simulink library "sm_wheel_loader_lib"  (R2025a)
settings: Solver=VariableStepAuto  StartTime=0.0  StopTime=10.0  RelTol=1e-3
undefined symbols (not defined in the file): AToTOrificeVector, BiPOrificeVector, boomHEArea, boomREArea, BToTOrificeVector, fluids, GRake, GToothL, GToothR, HMPST, HydFcnParams, logLoad, Position, PToAOrificeVector, PToBOrificeVector, RakeL, RakeR, testInput, Wheel_Loader, X, Y, Z
libraries: sm_lib x694, fl_lib x183, nesl_utility x74, SimscapeFluids_lib x62, sdl_lib x25, cvt_components_lib x25, simulink_extras x5, $bdroot x4, wheel_loader_contact_lib x4, ee_lib x2, SignalEditorBlockLib x1, batteryecm_lib x1
(part 11 of 26)

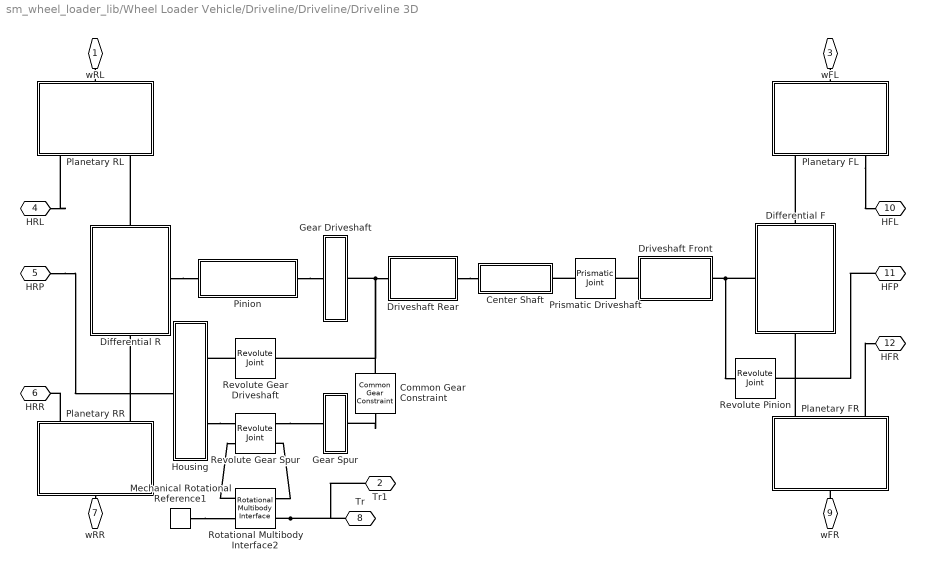
== system sm_wheel_loader_lib/Wheel Loader Vehicle/Driveline/Driveline/Driveline 3D ==
  Center Shaft : Subsystem
      mask Display: image('sm_wheel_loader_driveline_centerShaft_IMAGE.png');
  Common Gear Constraint : sm_lib/Gears and Couplings/Gears/Common Gear Constraint  GearType=External  SpecificationType=CenterDistanceRatio  CenterDistance=0.159173333333337  CenterDistanceUnits=m  GearRatio=60/34  BaseGearRadius=10.0  BaseGearRadiusUnits=cm  FollGearRadius=10.0  FollGearRadiusUnits=cm
  Differential F : Subsystem  mask{diff_casing_opc=HMPST.Vis.FDiffHou.opc}
      mask prompts: diff_casing_opc "Differential Casing Opacity (0-1)"
      settings: PortSchema="{\"entries\":[{\"content\":{\"sides\":[{\"content\":{\"connectorIds\":[\"LConn1\"]},\"type\":\"ConnectorPlacement.EquallySpacedRectSide\",\"uuid\":\"6caa8627-c586-4624-9941-b1de02eaac8c\"},{\"content\":{\"side\":\"RIGHT\"},\"type\":\"ConnectorPlacement.EquallySpacedRectSide\",\"uuid\":\"92f56e30-b0a7-4c10-9542-dd710977b4de\"},{\"content\":{\"connectorIds\":[\"LConn2\"],\"side\":\"TOP\"},\"type\":\"ConnectorPlacement.EquallySpacedRectSide\",\"uuid\":\"6e0658b9-6e92-4387-ac01-d2f307bfa341\"},{\"content\":{\"connectorIds\":[\"RConn1\"],\"side\":\"BOTTOM\"},\"type\":\"ConnectorPlacement.EquallySpacedRectSide\",\"uuid\":\"3080ce9a-db32-4b14-9c1c-37c42147fc35\"}]},\"type\":\"ConnectorPlacement.EquallySpacedConnector\",\"uuid\":\"9cd5bcd7-248c-4c6f-ba2a-fbf4d8f64778\"}],\"packageUris\":[\"http://schema.mathworks.com/mf0/Connector/R2020b\"],\"version\":\"1.0\"}"
      mask Display: image('sm_wheel_loader_Driveline3D_FDiff_IMAGE.png');
  Differential R : Subsystem  mask{diffR_casing_opc=HMPST.Vis.RDiffHou.opc}
      mask prompts: diffR_casing_opc "Differential Casing Opacity"
      settings: PortSchema="{\"entries\":[{\"content\":{\"sides\":[{\"content\":{\"connectorIds\":[\"LConn1\"]},\"type\":\"ConnectorPlacement.EquallySpacedRectSide\",\"uuid\":\"c6c34cb6-4adc-4dcc-9206-ba657dac7b98\"},{\"content\":{\"connectorIds\":[\"RConn1\"],\"side\":\"RIGHT\"},\"type\":\"ConnectorPlacement.EquallySpacedRectSide\",\"uuid\":\"746b050e-ecd9-4d25-a3bf-d6d079e98d03\"},{\"content\":{\"side\":\"TOP\"},\"type\":\"ConnectorPlacement.EquallySpacedRectSide\",\"uuid\":\"a331b284-bfab-47fb-9050-1886c295eab8\"},{\"content\":{\"connectorIds\":[\"RConn2\"],\"side\":\"BOTTOM\"},\"type\":\"ConnectorPlacement.EquallySpacedRectSide\",\"uuid\":\"57ab5774-feb0-4c3e-8c1c-741aef2b477c\"}]},\"type\":\"ConnectorPlacement.EquallySpacedConnector\",\"uuid\":\"0234f3ec-52d5-4d95-88b5-4fa84eea842c\"}],\"packageUris\":[\"http://schema.mathworks.com/mf0/Connector/R2020b\"],\"version\":\"1.0\"}"
      mask Display: image('sm_wheel_loader_Driveline3D_RDiff_IMAGE.png');
  Driveshaft Front : Subsystem  mask{popup_driveJointF=CV Joint}
      mask prompts: popup_driveJointF "Joint Type"
      mask init:
      | if(strcmp(get_param(gcb,'popup_driveJointF'),'CV Joint'))
      |     set_param([gcb '/Joint'],'LabelModeActiveChoice','CV_Joint');
      | else
      |     set_param([gcb '/Joint'],'LabelModeActiveChoice','U_Joint');
      | end
      settings: AttributesFormatString=%<popup_driveJointF>
      mask TypeOptions popup_driveJointF: CV Joint | U Joint
      mask Display:
      | if(strcmp(get_param(gcb,'popup_driveJointF'),'U Joint'))
      |     image('sm_wheel_loader_driveline_ujointF_IMAGE.png');
      | elseif(strcmp(get_param(gcb,'popup_driveJointF'),'CV Joint'))
      |     image('sm_wheel_loader_driveline_cvjointF_IMAGE.png');
      | end
  Driveshaft Rear : Subsystem  mask{popup_driveJointR=CV Joint}
      mask prompts: popup_driveJointR "Joint Type"
      mask init:
      | if(strcmp(get_param(gcb,'popup_driveJointR'),'CV Joint'))
      |     set_param([gcb '/Joint'],'LabelModeActiveChoice','CV_Joint');
      | else
      |     set_param([gcb '/Joint'],'LabelModeActiveChoice','U_Joint');
      | end
      settings: AttributesFormatString=%<popup_driveJointR>
      mask TypeOptions popup_driveJointR: CV Joint | U Joint
      mask Display:
      | if(strcmp(get_param(gcb,'popup_driveJointR'),'U Joint'))
      |     image('sm_wheel_loader_driveline_ujointR_IMAGE.png');
      | elseif(strcmp(get_param(gcb,'popup_driveJointR'),'CV Joint'))
      |     image('sm_wheel_loader_driveline_cvjointR_IMAGE.png');
      | end
  Gear Driveshaft : Subsystem  Tag=431AF5D6-54DA-7142-9431-C4596B630D74
      mask Display: image('sm_wheel_loader_driveline_gearDriveshaft_IMAGE.png')
  Gear Spur : Subsystem  Tag=6EB64544-2A1C-0847-BADC-74C9179BE488
      mask Display: image('sm_wheel_loader_driveline_gearSpur_IMAGE.png')
  Housing : Subsystem  Tag=FD1DF3FF-DA5A-0743-8F9C-61712535B657  mask{finalDr_casing_opc=HMPST.Vis.TfrGearHou.opc}
      mask prompts: finalDr_casing_opc "Final Drive Housing Opacity (0-1)"
      mask Display: image('sm_wheel_loader_driveline_gearHousing_IMAGE.png');
  Mechanical Rotational Reference1 : fl_lib/Mechanical/Rotational Elements/Mechanical Rotational Reference
  Pinion : Subsystem  Tag=8E104B94-12D7-814C-ADF4-87AC864C83F8
      mask Display: image('sm_wheel_loader_driveline_pinionR_IMAGE.png');
  Planetary FL : Subsystem  mask{casing_opc=HMPST.Vis.WhlPlaHou.opc}
      mask prompts: casing_opc "Casing Opacity (0-1)"
      mask Display: image('sm_wheel_loader_driveline_planetaryHubLtrans_IMAGE.png');
  Planetary FR : Subsystem  mask{casing_opc=HMPST.Vis.WhlPlaHou.opc}
      mask prompts: casing_opc "Casing Opacity (0-1)"
      mask Display: image('sm_wheel_loader_driveline_planetaryHubRtrans_IMAGE.png');
  Planetary RL : Subsystem  mask{casing_opc=HMPST.Vis.WhlPlaHou.opc}
      mask prompts: casing_opc "Casing Opacity (0-1)"
      mask Display: image('sm_wheel_loader_driveline_planetaryHubLtrans_IMAGE.png');
  Planetary RR : Subsystem  mask{casing_opc=HMPST.Vis.WhlPlaHou.opc}
      mask prompts: casing_opc "Casing Opacity (0-1)"
      mask Display: image('sm_wheel_loader_driveline_planetaryHubRtrans_IMAGE.png');
  Prismatic Driveshaft : sm_lib/Joints/Prismatic Joint  JointMode=Normal  CompositeWrenchDir=FollowerOnBase  CompositeWrenchFrame=BaseFrame  SenseConstraintForce=off  SenseConstraintTorque=off  SenseTotalForce=off  SenseTotalTorque=off  PositionTargetSpecify=off  PositionTargetPriority=High  PositionTargetValue=0  PositionTargetValueUnits=m  VelocityTargetSpecify=off  VelocityTargetPriority=High  VelocityTargetValue=0  VelocityTargetValueUnits=m/s  EquilibriumPosition=0  EquilibriumPositionUnits=m  SpringStiffness=0  SpringStiffnessUnits=N/m  DampingCoefficient=0  DampingCoefficientUnits=N/(m/s)  LowerLimitSpecify=off  LowerLimitBound=-1  LowerLimitBoundUnits=m  LowerLimitStiffness=1e6  LowerLimitStiffnessUnits=N/m  LowerLimitDamping=1e3  LowerLimitDampingUnits=N/(m/s)  LowerLimitTransitionRegionWidth=1e-4  LowerLimitTransitionRegionWidthUnits=m  UpperLimitSpecify=off  UpperLimitBound=1  UpperLimitBoundUnits=m  UpperLimitStiffness=1e6  UpperLimitStiffnessUnits=N/m  UpperLimitDamping=1e3  UpperLimitDampingUnits=N/(m/s)  UpperLimitTransitionRegionWidth=1e-4  UpperLimitTransitionRegionWidthUnits=m  TorqueActuationMode=NoTorque  MotionActuationMode=ComputedMotion  SensePosition=off  SenseVelocity=off  SenseAcceleration=off  SenseTorqueForce=off  SenseLowerLimitTorqueForce=off  SenseUpperLimitTorqueForce=off
  Revolute Gear Driveshaft : sm_lib/Joints/Revolute Joint  JointMode=Normal  CompositeWrenchDir=FollowerOnBase  CompositeWrenchFrame=BaseFrame  SenseConstraintForce=off  SenseConstraintTorque=off  SenseTotalForce=off  SenseTotalTorque=off  PositionTargetSpecify=off  PositionTargetPriority=High  PositionTargetValue=0  PositionTargetValueUnits=deg  VelocityTargetSpecify=off  VelocityTargetPriority=High  VelocityTargetValue=0  VelocityTargetValueUnits=deg/s  EquilibriumPosition=0  EquilibriumPositionUnits=deg  SpringStiffness=0  SpringStiffnessUnits=N*m/deg  DampingCoefficient=0  DampingCoefficientUnits=N*m/(deg/s)  LowerLimitSpecify=off  LowerLimitBound=-90  LowerLimitBoundUnits=deg  LowerLimitStiffness=1e4  LowerLimitStiffnessUnits=N*m/deg  LowerLimitDamping=10  LowerLimitDampingUnits=N*m/(deg/s)  LowerLimitTransitionRegionWidth=0.1  LowerLimitTransitionRegionWidthUnits=deg  UpperLimitSpecify=off  UpperLimitBound=90  UpperLimitBoundUnits=deg  UpperLimitStiffness=1e4  UpperLimitStiffnessUnits=N*m/deg  UpperLimitDamping=10  UpperLimitDampingUnits=N*m/(deg/s)  UpperLimitTransitionRegionWidth=0.1  UpperLimitTransitionRegionWidthUnits=deg  TorqueActuationMode=NoTorque  MotionActuationMode=ComputedMotion  SensePosition=off  SenseVelocity=off  SenseAcceleration=off  SenseTorqueForce=off  SenseLowerLimitTorqueForce=off  SenseUpperLimitTorqueForce=off
  Revolute Gear Spur : sm_lib/Joints/Revolute Joint  JointMode=Normal  CompositeWrenchDir=FollowerOnBase  CompositeWrenchFrame=BaseFrame  SenseConstraintForce=off  SenseConstraintTorque=off  SenseTotalForce=off  SenseTotalTorque=off  PositionTargetSpecify=off  PositionTargetPriority=High  PositionTargetValue=0  PositionTargetValueUnits=deg  VelocityTargetSpecify=off  VelocityTargetPriority=High  VelocityTargetValue=0  VelocityTargetValueUnits=deg/s  EquilibriumPosition=0  EquilibriumPositionUnits=deg  SpringStiffness=0  SpringStiffnessUnits=N*m/deg  DampingCoefficient=0  DampingCoefficientUnits=N*m/(deg/s)  LowerLimitSpecify=off  LowerLimitBound=-90  LowerLimitBoundUnits=deg  LowerLimitStiffness=1e4  LowerLimitStiffnessUnits=N*m/deg  LowerLimitDamping=10  LowerLimitDampingUnits=N*m/(deg/s)  LowerLimitTransitionRegionWidth=0.1  LowerLimitTransitionRegionWidthUnits=deg  UpperLimitSpecify=off  UpperLimitBound=90  UpperLimitBoundUnits=deg  UpperLimitStiffness=1e4  UpperLimitStiffnessUnits=N*m/deg  UpperLimitDamping=10  UpperLimitDampingUnits=N*m/(deg/s)  UpperLimitTransitionRegionWidth=0.1  UpperLimitTransitionRegionWidthUnits=deg  TorqueActuationMode=InputTorque  MotionActuationMode=ComputedMotion  SensePosition=off  SenseVelocity=on  SenseAcceleration=off  SenseTorqueForce=off  SenseLowerLimitTorqueForce=off  SenseUpperLimitTorqueForce=off
  Revolute Pinion : sm_lib/Joints/Revolute Joint  JointMode=Normal  CompositeWrenchDir=FollowerOnBase  CompositeWrenchFrame=BaseFrame  SenseConstraintForce=off  SenseConstraintTorque=off  SenseTotalForce=off  SenseTotalTorque=off  PositionTargetSpecify=off  PositionTargetPriority=High  PositionTargetValue=0  PositionTargetValueUnits=deg  VelocityTargetSpecify=off  VelocityTargetPriority=High  VelocityTargetValue=0  VelocityTargetValueUnits=deg/s  EquilibriumPosition=0  EquilibriumPositionUnits=deg  SpringStiffness=0  SpringStiffnessUnits=N*m/deg  DampingCoefficient=0  DampingCoefficientUnits=N*m/(deg/s)  LowerLimitSpecify=off  LowerLimitBound=-90  LowerLimitBoundUnits=deg  LowerLimitStiffness=1e4  LowerLimitStiffnessUnits=N*m/deg  LowerLimitDamping=10  LowerLimitDampingUnits=N*m/(deg/s)  LowerLimitTransitionRegionWidth=0.1  LowerLimitTransitionRegionWidthUnits=deg  UpperLimitSpecify=off  UpperLimitBound=90  UpperLimitBoundUnits=deg  UpperLimitStiffness=1e4  UpperLimitStiffnessUnits=N*m/deg  UpperLimitDamping=10  UpperLimitDampingUnits=N*m/(deg/s)  UpperLimitTransitionRegionWidth=0.1  UpperLimitTransitionRegionWidthUnits=deg  TorqueActuationMode=NoTorque  MotionActuationMode=ComputedMotion  SensePosition=off  SenseVelocity=off  SenseAcceleration=off  SenseTorqueForce=off  SenseLowerLimitTorqueForce=off  SenseUpperLimitTorqueForce=off
  Rotational Multibody Interface2 : fl_lib/Mechanical/Multibody Interfaces/Rotational Multibody Interface
  wRL : PMIOPort  Side=Left
  Tr1 : PMIOPort  Port=2  Side=Left
  wFL : PMIOPort  Port=3  Side=Left
  HRL : PMIOPort  Port=4  Side=Left
  HRP : PMIOPort  Port=5  Side=Left
  HRR : PMIOPort  Port=6  Side=Left
  wRR : PMIOPort  Port=7  Side=Right
  Tr : PMIOPort  Port=8  Side=Right
  wFR : PMIOPort  Port=9  Side=Right
  HFL : PMIOPort  Port=10  Side=Right
  HFP : PMIOPort  Port=11  Side=Right
  HFR : PMIOPort  Port=12  Side=Right
  connections:
  Prismatic Driveshaft/RConn1 -- Center Shaft/RConn1
  Driveshaft Rear/RConn1 -- Center Shaft/LConn1
  Planetary RL/LConn2 -- wRL/RConn1
  Planetary FL/RConn3 -- HFL/RConn1
  HFP/RConn1 -- Revolute Pinion/LConn1
  wFR/RConn1 -- Planetary FR/RConn2
  Planetary FL/LConn2 -- wFL/RConn1
  HRL/RConn1 -- Planetary RL/RConn1
  HRP/RConn1 -- Housing/LConn1
  Differential R/RConn2 -- Pinion/LConn1
  Planetary RR/RConn2 -- wRR/RConn1
  Rotational Multibody Interface2/RConn2 -- Tr1/RConn1 -- Tr/RConn1
  Planetary FR/LConn3 -- HFR/RConn1
  Planetary RR/LConn3 -- Differential R/RConn1
  Common Gear Constraint/LConn1 -- Gear Spur/RConn1
  Planetary RR/LConn1 -- HRR/RConn1
  Pinion/RConn1 -- Gear Driveshaft/RConn1
  Rotational Multibody Interface2/RConn1 -- Revolute Gear Spur/RConn2
  Rotational Multibody Interface2/LConn1 -- Revolute Gear Spur/LConn2
  Mechanical Rotational Reference1/LConn1 -- Rotational Multibody Interface2/LConn2
  Driveshaft Front/LConn1 -- Prismatic Driveshaft/LConn1
  Revolute Gear Spur/RConn1 -- Gear Spur/LConn1
  Differential F/LConn2 -- Planetary FL/RConn1
  Revolute Gear Driveshaft/LConn1 -- Housing/RConn1
  Driveshaft Front/RConn1 -- Revolute Pinion/RConn1 -- Differential F/LConn1
  Driveshaft Rear/LConn1 -- Gear Driveshaft/LConn1 -- Revolute Gear Driveshaft/RConn1 -- Common Gear Constraint/RConn1
  Planetary FR/LConn1 -- Differential F/RConn1
  Housing/RConn2 -- Revolute Gear Spur/LConn1
  Differential R/LConn1 -- Planetary RL/RConn3

== system sm_wheel_loader_lib/Wheel Loader Vehicle/Driveline/Wheel FL/Hub ==
  Bolts : sm_lib/Body Elements/File Solid  ExtGeomFileName=WheelFL_Hub_Bolts.STEP  UnitType=FromFile  ExtGeomFileUnits=m  StepReaderType=HEX  ExportConvexHullGeometry=off  InertiaType=Custom  BasedOnType=DensityFromFile  Density=1000  DensityUnits=kg/m^3  Mass=Wheel_Loader.bodyGroups(33).subGroups(2).inertialProperties.mass  MassUnits=kg  CenterOfMass=Wheel_Loader.bodyGroups(33).subGroups(2).inertialProperties.centerOfMass  CenterOfMassUnits=m  MomentsOfInertia=Wheel_Loader.bodyGroups(33).subGroups(2).inertialProperties.momentsOfInertia  MomentsOfInertiaUnits=kg*m^2  ProductsOfInertia=Wheel_Loader.bodyGroups(33).subGroups(2).inertialProperties.productsOfInertia  ProductsOfInertiaUnits=kg*m^2  GraphicType=FromGeometry  MarkerShape=Sphere  MarkerSize=10  GraphicVisPropType=SimpleVisualProperties  GraphicDiffuseColor=Wheel_Loader.bodyGroups(33).subGroups(2).visualProperties.rgb  GraphicOpacity=Wheel_Loader.bodyGroups(33).subGroups(2).visualProperties.opacity  GraphicSpecularColor=[0.5 0.5 0.5 1.0]  GraphicAmbientColor=[0.15 0.15 0.15 1.0]  GraphicEmissiveColor=[0.0 0.0 0.0 1.0]  GraphicShininess=75  DoExposeReferenceFrame=on  SerializedFrames=<Frames/>
  Hub : sm_lib/Body Elements/File Solid  ExtGeomFileName=WheelFL_Hub.STEP  UnitType=FromFile  ExtGeomFileUnits=m  StepReaderType=HEX  ExportConvexHullGeometry=off  InertiaType=Custom  BasedOnType=DensityFromFile  Density=1000  DensityUnits=kg/m^3  Mass=Wheel_Loader.bodyGroups(33).subGroups(1).inertialProperties.mass  MassUnits=kg  CenterOfMass=Wheel_Loader.bodyGroups(33).subGroups(1).inertialProperties.centerOfMass  CenterOfMassUnits=m  MomentsOfInertia=Wheel_Loader.bodyGroups(33).subGroups(1).inertialProperties.momentsOfInertia  MomentsOfInertiaUnits=kg*m^2  ProductsOfInertia=Wheel_Loader.bodyGroups(33).subGroups(1).inertialProperties.productsOfInertia  ProductsOfInertiaUnits=kg*m^2  GraphicType=FromGeometry  MarkerShape=Sphere  MarkerSize=10  GraphicVisPropType=SimpleVisualProperties  GraphicDiffuseColor=Wheel_Loader.bodyGroups(33).subGroups(1).visualProperties.rgb  GraphicOpacity=Wheel_Loader.bodyGroups(33).subGroups(1).visualProperties.opacity  GraphicSpecularColor=[0.5 0.5 0.5 1.0]  GraphicAmbientColor=[0.15 0.15 0.15 1.0]  GraphicEmissiveColor=[0.0 0.0 0.0 1.0]  GraphicShininess=75  DoExposeReferenceFrame=on  SerializedFrames=<Frames/>
  RT_LFFDCarrier_LFWheelHub_Weld : sm_lib/Frames and Transforms/Rigid Transform  RotationMethod=RotationMatrix  FollAlignAxisA=+X  BaseAlignAxisA=+Y  FollAlignAxisB=+Y  BaseAlignAxisB=+Z  RotationStandardAxis=+Z  RotationAngle=0.0  RotationAngleUnits=deg  RotationArbitraryAxis=[0 0 1]  RotationSequenceAxes=FollowerAxes  RotationSequence=XYX  RotationSequenceAngles=[0 0 0]  RotationSequenceAnglesUnits=deg  RotationMatrix=Wheel_Loader.coordSys(70).transform.rotation  Quaternion=[1 0 0 0]  TranslationMethod=Cartesian  TranslationCartesianOffset=Wheel_Loader.coordSys(70).transform.translation  TranslationCartesianOffsetUnits=m  TranslationStandardAxis=+Z  TranslationStandardOffset=0  TranslationStandardOffsetUnits=m  TranslationROffset=0  TranslationROffsetUnits=m  TranslationThetaOffset=0  TranslationThetaOffsetUnits=deg  TranslationZOffset=0  TranslationZOffsetUnits=m
  RT_LF_WheelHub_Tire_Weld : sm_lib/Frames and Transforms/Rigid Transform  RotationMethod=RotationMatrix  FollAlignAxisA=+X  BaseAlignAxisA=+Y  FollAlignAxisB=+Y  BaseAlignAxisB=+Z  RotationStandardAxis=+Z  RotationAngle=0.0  RotationAngleUnits=deg  RotationArbitraryAxis=[0 0 1]  RotationSequenceAxes=FollowerAxes  RotationSequence=XYX  RotationSequenceAngles=[0 0 0]  RotationSequenceAnglesUnits=deg  RotationMatrix=Wheel_Loader.coordSys(39).transform.rotation  Quaternion=[1 0 0 0]  TranslationMethod=Cartesian  TranslationCartesianOffset=Wheel_Loader.coordSys(39).transform.translation  TranslationCartesianOffsetUnits=m  TranslationStandardAxis=+Z  TranslationStandardOffset=0  TranslationStandardOffsetUnits=m  TranslationROffset=0  TranslationROffsetUnits=m  TranslationThetaOffset=0  TranslationThetaOffsetUnits=deg  TranslationZOffset=0  TranslationZOffsetUnits=m
  Transform Center Offset : sm_lib/Frames and Transforms/Rigid Transform  RotationMethod=None  FollAlignAxisA=+X  BaseAlignAxisA=+Y  FollAlignAxisB=+Y  BaseAlignAxisB=+Z  RotationStandardAxis=+Z  RotationAngle=0.0  RotationAngleUnits=deg  RotationArbitraryAxis=[0 0 1]  RotationSequenceAxes=FollowerAxes  RotationSequence=XYX  RotationSequenceAngles=[0 0 0]  RotationSequenceAnglesUnits=deg  RotationMatrix=[1 0 0; 0 1 0; 0 0 1]  Quaternion=[1 0 0 0]  TranslationMethod=Cartesian  TranslationCartesianOffset="-[0.000007750824851   0.000006230422858 0]"  TranslationCartesianOffsetUnits=m  TranslationStandardAxis=+Z  TranslationStandardOffset=0  TranslationStandardOffsetUnits=m  TranslationROffset=0  TranslationROffsetUnits=m  TranslationThetaOffset=0  TranslationThetaOffsetUnits=deg  TranslationZOffset=0  TranslationZOffsetUnits=m
  B1 : PMIOPort  Side=Left
  F1 : PMIOPort  Port=2  Side=Right
  connections:
  Transform Center Offset/RConn1 -- F1/RConn1
  RT_LFFDCarrier_LFWheelHub_Weld/RConn1 -- B1/RConn1
  RT_LF_WheelHub_Tire_Weld/LConn1 -- RT_LFFDCarrier_LFWheelHub_Weld/LConn1 -- Hub/RConn1 -- Bolts/RConn1
  RT_LF_WheelHub_Tire_Weld/RConn1 -- Transform Center Offset/LConn1

== system sm_wheel_loader_lib/Wheel Loader Vehicle/Driveline/Wheel FL/Tire ==
  RT_Gnd_LFTire : sm_lib/Frames and Transforms/Rigid Transform  RotationMethod=RotationMatrix  FollAlignAxisA=+X  BaseAlignAxisA=+Y  FollAlignAxisB=+Y  BaseAlignAxisB=+Z  RotationStandardAxis=+Z  RotationAngle=0.0  RotationAngleUnits=deg  RotationArbitraryAxis=[0 0 1]  RotationSequenceAxes=FollowerAxes  RotationSequence=XYX  RotationSequenceAngles=[0 0 0]  RotationSequenceAnglesUnits=deg  RotationMatrix=Wheel_Loader.coordSys(39).transform.rotation  Quaternion=[1 0 0 0]  TranslationMethod=Cartesian  TranslationCartesianOffset=Wheel_Loader.coordSys(39).transform.translation  TranslationCartesianOffsetUnits=m  TranslationStandardAxis=+Z  TranslationStandardOffset=0  TranslationStandardOffsetUnits=m  TranslationROffset=0  TranslationROffsetUnits=m  TranslationThetaOffset=0  TranslationThetaOffsetUnits=deg  TranslationZOffset=0  TranslationZOffsetUnits=m
  RT_LF_WheelHub_Tire_Weld : sm_lib/Frames and Transforms/Rigid Transform  RotationMethod=RotationMatrix  FollAlignAxisA=+X  BaseAlignAxisA=+Y  FollAlignAxisB=+Y  BaseAlignAxisB=+Z  RotationStandardAxis=+Z  RotationAngle=0.0  RotationAngleUnits=deg  RotationArbitraryAxis=[0 0 1]  RotationSequenceAxes=FollowerAxes  RotationSequence=XYX  RotationSequenceAngles=[0 0 0]  RotationSequenceAnglesUnits=deg  RotationMatrix=Wheel_Loader.coordSys(39).transform.rotation  Quaternion=[1 0 0 0]  TranslationMethod=Cartesian  TranslationCartesianOffset=Wheel_Loader.coordSys(39).transform.translation  TranslationCartesianOffsetUnits=m  TranslationStandardAxis=+Z  TranslationStandardOffset=0  TranslationStandardOffsetUnits=m  TranslationROffset=0  TranslationROffsetUnits=m  TranslationThetaOffset=0  TranslationThetaOffsetUnits=deg  TranslationZOffset=0  TranslationZOffsetUnits=m
  Tire : sm_lib/Body Elements/File Solid  ExtGeomFileName=WheelFL_Tire.STEP  UnitType=FromFile  ExtGeomFileUnits=m  StepReaderType=HEX  ExportConvexHullGeometry=off  InertiaType=Custom  BasedOnType=DensityFromFile  Density=1000  DensityUnits=kg/m^3  Mass=Wheel_Loader.bodyGroups(25).subGroups(1).inertialProperties.mass  MassUnits=kg  CenterOfMass="Wheel_Loader.bodyGroups(25).subGroups(1).inertialProperties.centerOfMass-[0 0.511868381902759  -0.664959371798891]'*1e-5"  CenterOfMassUnits=m  MomentsOfInertia=Wheel_Loader.bodyGroups(25).subGroups(1).inertialProperties.momentsOfInertia  MomentsOfInertiaUnits=kg*m^2  ProductsOfInertia=Wheel_Loader.bodyGroups(25).subGroups(1).inertialProperties.productsOfInertia  ProductsOfInertiaUnits=kg*m^2  GraphicType=FromGeometry  MarkerShape=Sphere  MarkerSize=10  GraphicVisPropType=SimpleVisualProperties  GraphicDiffuseColor=Wheel_Loader.bodyGroups(25).subGroups(1).visualProperties.rgb  GraphicOpacity=Wheel_Loader.bodyGroups(25).subGroups(1).visualProperties.opacity  GraphicSpecularColor=[0.5 0.5 0.5 1.0]  GraphicAmbientColor=[0.15 0.15 0.15 1.0]  GraphicEmissiveColor=[0.0 0.0 0.0 1.0]  GraphicShininess=75  DoExposeReferenceFrame=on  SerializedFrames=<Frames/>
  B1 : PMIOPort  Side=Left
  B2 : PMIOPort  Port=2  Side=Right
  connections:
  Tire/RConn1 -- RT_LF_WheelHub_Tire_Weld/LConn1 -- RT_Gnd_LFTire/LConn1
  RT_LF_WheelHub_Tire_Weld/RConn1 -- B1/RConn1
  RT_Gnd_LFTire/RConn1 -- B2/RConn1

== system sm_wheel_loader_lib/Wheel Loader Vehicle/Driveline/Wheel FR/Hub ==
  Bolts : sm_lib/Body Elements/File Solid  ExtGeomFileName=WheelFR_Hub_Bolts.STEP  UnitType=FromFile  ExtGeomFileUnits=m  StepReaderType=HEX  ExportConvexHullGeometry=off  InertiaType=Custom  BasedOnType=DensityFromFile  Density=1000  DensityUnits=kg/m^3  Mass=Wheel_Loader.bodyGroups(32).subGroups(2).inertialProperties.mass  MassUnits=kg  CenterOfMass=Wheel_Loader.bodyGroups(32).subGroups(2).inertialProperties.centerOfMass  CenterOfMassUnits=m  MomentsOfInertia=Wheel_Loader.bodyGroups(32).subGroups(2).inertialProperties.momentsOfInertia  MomentsOfInertiaUnits=kg*m^2  ProductsOfInertia=Wheel_Loader.bodyGroups(32).subGroups(2).inertialProperties.productsOfInertia  ProductsOfInertiaUnits=kg*m^2  GraphicType=FromGeometry  MarkerShape=Sphere  MarkerSize=10  GraphicVisPropType=SimpleVisualProperties  GraphicDiffuseColor=Wheel_Loader.bodyGroups(32).subGroups(2).visualProperties.rgb  GraphicOpacity=Wheel_Loader.bodyGroups(32).subGroups(2).visualProperties.opacity  GraphicSpecularColor=[0.5 0.5 0.5 1.0]  GraphicAmbientColor=[0.15 0.15 0.15 1.0]  GraphicEmissiveColor=[0.0 0.0 0.0 1.0]  GraphicShininess=75  DoExposeReferenceFrame=on  SerializedFrames=<Frames/>
  Hub : sm_lib/Body Elements/File Solid  ExtGeomFileName=WheelFR_Hub.STEP  UnitType=FromFile  ExtGeomFileUnits=m  StepReaderType=HEX  ExportConvexHullGeometry=off  InertiaType=Custom  BasedOnType=DensityFromFile  Density=1000  DensityUnits=kg/m^3  Mass=Wheel_Loader.bodyGroups(32).subGroups(1).inertialProperties.mass  MassUnits=kg  CenterOfMass=Wheel_Loader.bodyGroups(32).subGroups(1).inertialProperties.centerOfMass  CenterOfMassUnits=m  MomentsOfInertia=Wheel_Loader.bodyGroups(32).subGroups(1).inertialProperties.momentsOfInertia  MomentsOfInertiaUnits=kg*m^2  ProductsOfInertia=Wheel_Loader.bodyGroups(32).subGroups(1).inertialProperties.productsOfInertia  ProductsOfInertiaUnits=kg*m^2  GraphicType=FromGeometry  MarkerShape=Sphere  MarkerSize=10  GraphicVisPropType=SimpleVisualProperties  GraphicDiffuseColor=Wheel_Loader.bodyGroups(32).subGroups(1).visualProperties.rgb  GraphicOpacity=Wheel_Loader.bodyGroups(32).subGroups(1).visualProperties.opacity  GraphicSpecularColor=[0.5 0.5 0.5 1.0]  GraphicAmbientColor=[0.15 0.15 0.15 1.0]  GraphicEmissiveColor=[0.0 0.0 0.0 1.0]  GraphicShininess=75  DoExposeReferenceFrame=on  SerializedFrames=<Frames/>
  RT_RFFDCarrier_RFWheelHub_Weld : sm_lib/Frames and Transforms/Rigid Transform  RotationMethod=RotationMatrix  FollAlignAxisA=+X  BaseAlignAxisA=+Y  FollAlignAxisB=+Y  BaseAlignAxisB=+Z  RotationStandardAxis=+Z  RotationAngle=0.0  RotationAngleUnits=deg  RotationArbitraryAxis=[0 0 1]  RotationSequenceAxes=FollowerAxes  RotationSequence=XYX  RotationSequenceAngles=[0 0 0]  RotationSequenceAnglesUnits=deg  RotationMatrix=Wheel_Loader.coordSys(66).transform.rotation  Quaternion=[1 0 0 0]  TranslationMethod=Cartesian  TranslationCartesianOffset=Wheel_Loader.coordSys(66).transform.translation  TranslationCartesianOffsetUnits=m  TranslationStandardAxis=+Z  TranslationStandardOffset=0  TranslationStandardOffsetUnits=m  TranslationROffset=0  TranslationROffsetUnits=m  TranslationThetaOffset=0  TranslationThetaOffsetUnits=deg  TranslationZOffset=0  TranslationZOffsetUnits=m
  RT_RF_WheelHub_Tire_Weld : sm_lib/Frames and Transforms/Rigid Transform  RotationMethod=RotationMatrix  FollAlignAxisA=+X  BaseAlignAxisA=+Y  FollAlignAxisB=+Y  BaseAlignAxisB=+Z  RotationStandardAxis=+Z  RotationAngle=0.0  RotationAngleUnits=deg  RotationArbitraryAxis=[0 0 1]  RotationSequenceAxes=FollowerAxes  RotationSequence=XYX  RotationSequenceAngles=[0 0 0]  RotationSequenceAnglesUnits=deg  RotationMatrix=Wheel_Loader.coordSys(40).transform.rotation  Quaternion=[1 0 0 0]  TranslationMethod=Cartesian  TranslationCartesianOffset=Wheel_Loader.coordSys(40).transform.translation  TranslationCartesianOffsetUnits=m  TranslationStandardAxis=+Z  TranslationStandardOffset=0  TranslationStandardOffsetUnits=m  TranslationROffset=0  TranslationROffsetUnits=m  TranslationThetaOffset=0  TranslationThetaOffsetUnits=deg  TranslationZOffset=0  TranslationZOffsetUnits=m
  Transform Center Offset : sm_lib/Frames and Transforms/Rigid Transform  RotationMethod=None  FollAlignAxisA=+X  BaseAlignAxisA=+Y  FollAlignAxisB=+Y  BaseAlignAxisB=+Z  RotationStandardAxis=+Z  RotationAngle=0.0  RotationAngleUnits=deg  RotationArbitraryAxis=[0 0 1]  RotationSequenceAxes=FollowerAxes  RotationSequence=XYX  RotationSequenceAngles=[0 0 0]  RotationSequenceAnglesUnits=deg  RotationMatrix=[1 0 0; 0 1 0; 0 0 1]  Quaternion=[1 0 0 0]  TranslationMethod=Cartesian  TranslationCartesianOffset="-[0.000002607460598  0.000009596593759 0]"  TranslationCartesianOffsetUnits=m  TranslationStandardAxis=+Z  TranslationStandardOffset=0  TranslationStandardOffsetUnits=m  TranslationROffset=0  TranslationROffsetUnits=m  TranslationThetaOffset=0  TranslationThetaOffsetUnits=deg  TranslationZOffset=0  TranslationZOffsetUnits=m
  B1 : PMIOPort  Side=Left
  F1 : PMIOPort  Port=2  Side=Right
  connections:
  RT_RF_WheelHub_Tire_Weld/RConn1 -- Transform Center Offset/LConn1
  RT_RFFDCarrier_RFWheelHub_Weld/RConn1 -- B1/RConn1
  Hub/RConn1 -- RT_RF_WheelHub_Tire_Weld/LConn1 -- RT_RFFDCarrier_RFWheelHub_Weld/LConn1 -- Bolts/RConn1
  Transform Center Offset/RConn1 -- F1/RConn1

== system sm_wheel_loader_lib/Wheel Loader Vehicle/Driveline/Wheel FR/Tire ==
  RT_Gnd_RFTire : sm_lib/Frames and Transforms/Rigid Transform  RotationMethod=RotationMatrix  FollAlignAxisA=+X  BaseAlignAxisA=+Y  FollAlignAxisB=+Y  BaseAlignAxisB=+Z  RotationStandardAxis=+Z  RotationAngle=0.0  RotationAngleUnits=deg  RotationArbitraryAxis=[0 0 1]  RotationSequenceAxes=FollowerAxes  RotationSequence=XYX  RotationSequenceAngles=[0 0 0]  RotationSequenceAnglesUnits=deg  RotationMatrix=Wheel_Loader.coordSys(40).transform.rotation  Quaternion=[1 0 0 0]  TranslationMethod=Cartesian  TranslationCartesianOffset=Wheel_Loader.coordSys(40).transform.translation  TranslationCartesianOffsetUnits=m  TranslationStandardAxis=+Z  TranslationStandardOffset=0  TranslationStandardOffsetUnits=m  TranslationROffset=0  TranslationROffsetUnits=m  TranslationThetaOffset=0  TranslationThetaOffsetUnits=deg  TranslationZOffset=0  TranslationZOffsetUnits=m
  RT_RF_WheelHub_Tire_Weld : sm_lib/Frames and Transforms/Rigid Transform  RotationMethod=RotationMatrix  FollAlignAxisA=+X  BaseAlignAxisA=+Y  FollAlignAxisB=+Y  BaseAlignAxisB=+Z  RotationStandardAxis=+Z  RotationAngle=0.0  RotationAngleUnits=deg  RotationArbitraryAxis=[0 0 1]  RotationSequenceAxes=FollowerAxes  RotationSequence=XYX  RotationSequenceAngles=[0 0 0]  RotationSequenceAnglesUnits=deg  RotationMatrix=Wheel_Loader.coordSys(40).transform.rotation  Quaternion=[1 0 0 0]  TranslationMethod=Cartesian  TranslationCartesianOffset=Wheel_Loader.coordSys(40).transform.translation  TranslationCartesianOffsetUnits=m  TranslationStandardAxis=+Z  TranslationStandardOffset=0  TranslationStandardOffsetUnits=m  TranslationROffset=0  TranslationROffsetUnits=m  TranslationThetaOffset=0  TranslationThetaOffsetUnits=deg  TranslationZOffset=0  TranslationZOffsetUnits=m
  Tire : sm_lib/Body Elements/File Solid  ExtGeomFileName=WheelFR_Tire.STEP  UnitType=FromFile  ExtGeomFileUnits=m  StepReaderType=HEX  ExportConvexHullGeometry=off  InertiaType=Custom  BasedOnType=DensityFromFile  Density=1000  DensityUnits=kg/m^3  Mass=Wheel_Loader.bodyGroups(24).subGroups(1).inertialProperties.mass  MassUnits=kg  CenterOfMass="Wheel_Loader.bodyGroups(24).subGroups(1).inertialProperties.centerOfMass-[0 0.803543223093507  -0.271445672600512]'*1e-5"  CenterOfMassUnits=m  MomentsOfInertia=Wheel_Loader.bodyGroups(24).subGroups(1).inertialProperties.momentsOfInertia  MomentsOfInertiaUnits=kg*m^2  ProductsOfInertia=Wheel_Loader.bodyGroups(24).subGroups(1).inertialProperties.productsOfInertia  ProductsOfInertiaUnits=kg*m^2  GraphicType=FromGeometry  MarkerShape=Sphere  MarkerSize=10  GraphicVisPropType=SimpleVisualProperties  GraphicDiffuseColor=Wheel_Loader.bodyGroups(24).subGroups(1).visualProperties.rgb  GraphicOpacity=Wheel_Loader.bodyGroups(24).subGroups(1).visualProperties.opacity  GraphicSpecularColor=[0.5 0.5 0.5 1.0]  GraphicAmbientColor=[0.15 0.15 0.15 1.0]  GraphicEmissiveColor=[0.0 0.0 0.0 1.0]  GraphicShininess=75  DoExposeReferenceFrame=on  SerializedFrames=<Frames/>
  B1 : PMIOPort  Side=Left
  B2 : PMIOPort  Port=2  Side=Right
  connections:
  RT_Gnd_RFTire/RConn1 -- B2/RConn1
  RT_RF_WheelHub_Tire_Weld/RConn1 -- B1/RConn1
  RT_Gnd_RFTire/LConn1 -- RT_RF_WheelHub_Tire_Weld/LConn1 -- Tire/RConn1

== system sm_wheel_loader_lib/Wheel Loader Vehicle/Driveline/Wheel RL/Hub ==
  Bolts : sm_lib/Body Elements/File Solid  ExtGeomFileName=WheelRL_Hub_Bolts.STEP  UnitType=FromFile  ExtGeomFileUnits=m  StepReaderType=HEX  ExportConvexHullGeometry=off  InertiaType=Custom  BasedOnType=DensityFromFile  Density=1000  DensityUnits=kg/m^3  Mass=Wheel_Loader.bodyGroups(35).subGroups(2).inertialProperties.mass  MassUnits=kg  CenterOfMass=Wheel_Loader.bodyGroups(35).subGroups(2).inertialProperties.centerOfMass  CenterOfMassUnits=m  MomentsOfInertia=Wheel_Loader.bodyGroups(35).subGroups(2).inertialProperties.momentsOfInertia  MomentsOfInertiaUnits=kg*m^2  ProductsOfInertia=Wheel_Loader.bodyGroups(35).subGroups(2).inertialProperties.productsOfInertia  ProductsOfInertiaUnits=kg*m^2  GraphicType=FromGeometry  MarkerShape=Sphere  MarkerSize=10  GraphicVisPropType=SimpleVisualProperties  GraphicDiffuseColor=Wheel_Loader.bodyGroups(35).subGroups(2).visualProperties.rgb  GraphicOpacity=Wheel_Loader.bodyGroups(35).subGroups(2).visualProperties.opacity  GraphicSpecularColor=[0.5 0.5 0.5 1.0]  GraphicAmbientColor=[0.15 0.15 0.15 1.0]  GraphicEmissiveColor=[0.0 0.0 0.0 1.0]  GraphicShininess=75  DoExposeReferenceFrame=on  SerializedFrames=<Frames/>
  Hub : sm_lib/Body Elements/File Solid  ExtGeomFileName=WheelRL_Hub.STEP  UnitType=FromFile  ExtGeomFileUnits=m  StepReaderType=HEX  ExportConvexHullGeometry=off  InertiaType=Custom  BasedOnType=DensityFromFile  Density=1000  DensityUnits=kg/m^3  Mass=Wheel_Loader.bodyGroups(35).subGroups(1).inertialProperties.mass  MassUnits=kg  CenterOfMass=Wheel_Loader.bodyGroups(35).subGroups(1).inertialProperties.centerOfMass  CenterOfMassUnits=m  MomentsOfInertia=Wheel_Loader.bodyGroups(35).subGroups(1).inertialProperties.momentsOfInertia  MomentsOfInertiaUnits=kg*m^2  ProductsOfInertia=Wheel_Loader.bodyGroups(35).subGroups(1).inertialProperties.productsOfInertia  ProductsOfInertiaUnits=kg*m^2  GraphicType=FromGeometry  MarkerShape=Sphere  MarkerSize=10  GraphicVisPropType=SimpleVisualProperties  GraphicDiffuseColor=Wheel_Loader.bodyGroups(35).subGroups(1).visualProperties.rgb  GraphicOpacity=Wheel_Loader.bodyGroups(35).subGroups(1).visualProperties.opacity  GraphicSpecularColor=[0.5 0.5 0.5 1.0]  GraphicAmbientColor=[0.15 0.15 0.15 1.0]  GraphicEmissiveColor=[0.0 0.0 0.0 1.0]  GraphicShininess=75  DoExposeReferenceFrame=on  SerializedFrames=<Frames/>
  RT_LRFDCarrier_LRWheelHub_Weld : sm_lib/Frames and Transforms/Rigid Transform  RotationMethod=RotationMatrix  FollAlignAxisA=+X  BaseAlignAxisA=+Y  FollAlignAxisB=+Y  BaseAlignAxisB=+Z  RotationStandardAxis=+Z  RotationAngle=0.0  RotationAngleUnits=deg  RotationArbitraryAxis=[0 0 1]  RotationSequenceAxes=FollowerAxes  RotationSequence=XYX  RotationSequenceAngles=[0 0 0]  RotationSequenceAnglesUnits=deg  RotationMatrix=Wheel_Loader.coordSys(62).transform.rotation  Quaternion=[1 0 0 0]  TranslationMethod=Cartesian  TranslationCartesianOffset=Wheel_Loader.coordSys(62).transform.translation  TranslationCartesianOffsetUnits=m  TranslationStandardAxis=+Z  TranslationStandardOffset=0  TranslationStandardOffsetUnits=m  TranslationROffset=0  TranslationROffsetUnits=m  TranslationThetaOffset=0  TranslationThetaOffsetUnits=deg  TranslationZOffset=0  TranslationZOffsetUnits=m
  RT_LR_WheelHub_Tire_Weld : sm_lib/Frames and Transforms/Rigid Transform  RotationMethod=RotationMatrix  FollAlignAxisA=+X  BaseAlignAxisA=+Y  FollAlignAxisB=+Y  BaseAlignAxisB=+Z  RotationStandardAxis=+Z  RotationAngle=0.0  RotationAngleUnits=deg  RotationArbitraryAxis=[0 0 1]  RotationSequenceAxes=FollowerAxes  RotationSequence=XYX  RotationSequenceAngles=[0 0 0]  RotationSequenceAnglesUnits=deg  RotationMatrix=Wheel_Loader.coordSys(41).transform.rotation  Quaternion=[1 0 0 0]  TranslationMethod=Cartesian  TranslationCartesianOffset=Wheel_Loader.coordSys(41).transform.translation  TranslationCartesianOffsetUnits=m  TranslationStandardAxis=+Z  TranslationStandardOffset=0  TranslationStandardOffsetUnits=m  TranslationROffset=0  TranslationROffsetUnits=m  TranslationThetaOffset=0  TranslationThetaOffsetUnits=deg  TranslationZOffset=0  TranslationZOffsetUnits=m
  Rigid Transform : sm_lib/Frames and Transforms/Rigid Transform  RotationMethod=None  FollAlignAxisA=+X  BaseAlignAxisA=+Y  FollAlignAxisB=+Y  BaseAlignAxisB=+Z  RotationStandardAxis=+Z  RotationAngle=0.0  RotationAngleUnits=deg  RotationArbitraryAxis=[0 0 1]  RotationSequenceAxes=FollowerAxes  RotationSequence=XYX  RotationSequenceAngles=[0 0 0]  RotationSequenceAnglesUnits=deg  RotationMatrix=[1 0 0; 0 1 0; 0 0 1]  Quaternion=[1 0 0 0]  TranslationMethod=Cartesian  TranslationCartesianOffset="-[-0.000001165128093  -0.000009876028086 0]"  TranslationCartesianOffsetUnits=m  TranslationStandardAxis=+Z  TranslationStandardOffset=0  TranslationStandardOffsetUnits=m  TranslationROffset=0  TranslationROffsetUnits=m  TranslationThetaOffset=0  TranslationThetaOffsetUnits=deg  TranslationZOffset=0  TranslationZOffsetUnits=m
  B1 : PMIOPort  Side=Left
  F1 : PMIOPort  Port=2  Side=Right
  connections:
  RT_LR_WheelHub_Tire_Weld/RConn1 -- Rigid Transform/LConn1
  RT_LRFDCarrier_LRWheelHub_Weld/RConn1 -- B1/RConn1
  Hub/RConn1 -- RT_LR_WheelHub_Tire_Weld/LConn1 -- RT_LRFDCarrier_LRWheelHub_Weld/LConn1 -- Bolts/RConn1
  Rigid Transform/RConn1 -- F1/RConn1

== system sm_wheel_loader_lib/Wheel Loader Vehicle/Driveline/Wheel RL/Tire ==
  RT_Gnd_LRTire : sm_lib/Frames and Transforms/Rigid Transform  RotationMethod=RotationMatrix  FollAlignAxisA=+X  BaseAlignAxisA=+Y  FollAlignAxisB=+Y  BaseAlignAxisB=+Z  RotationStandardAxis=+Z  RotationAngle=0.0  RotationAngleUnits=deg  RotationArbitraryAxis=[0 0 1]  RotationSequenceAxes=FollowerAxes  RotationSequence=XYX  RotationSequenceAngles=[0 0 0]  RotationSequenceAnglesUnits=deg  RotationMatrix=Wheel_Loader.coordSys(41).transform.rotation  Quaternion=[1 0 0 0]  TranslationMethod=Cartesian  TranslationCartesianOffset=Wheel_Loader.coordSys(41).transform.translation  TranslationCartesianOffsetUnits=m  TranslationStandardAxis=+Z  TranslationStandardOffset=0  TranslationStandardOffsetUnits=m  TranslationROffset=0  TranslationROffsetUnits=m  TranslationThetaOffset=0  TranslationThetaOffsetUnits=deg  TranslationZOffset=0  TranslationZOffsetUnits=m
  RT_LR_WheelHub_Tire_Weld : sm_lib/Frames and Transforms/Rigid Transform  RotationMethod=RotationMatrix  FollAlignAxisA=+X  BaseAlignAxisA=+Y  FollAlignAxisB=+Y  BaseAlignAxisB=+Z  RotationStandardAxis=+Z  RotationAngle=0.0  RotationAngleUnits=deg  RotationArbitraryAxis=[0 0 1]  RotationSequenceAxes=FollowerAxes  RotationSequence=XYX  RotationSequenceAngles=[0 0 0]  RotationSequenceAnglesUnits=deg  RotationMatrix=Wheel_Loader.coordSys(41).transform.rotation  Quaternion=[1 0 0 0]  TranslationMethod=Cartesian  TranslationCartesianOffset=Wheel_Loader.coordSys(41).transform.translation  TranslationCartesianOffsetUnits=m  TranslationStandardAxis=+Z  TranslationStandardOffset=0  TranslationStandardOffsetUnits=m  TranslationROffset=0  TranslationROffsetUnits=m  TranslationThetaOffset=0  TranslationThetaOffsetUnits=deg  TranslationZOffset=0  TranslationZOffsetUnits=m
  Tire : sm_lib/Body Elements/File Solid  ExtGeomFileName=WheelRL_Tire.STEP  UnitType=FromFile  ExtGeomFileUnits=m  StepReaderType=HEX  ExportConvexHullGeometry=off  InertiaType=Custom  BasedOnType=DensityFromFile  Density=1000  DensityUnits=kg/m^3  Mass=Wheel_Loader.bodyGroups(27).subGroups(1).inertialProperties.mass  MassUnits=kg  CenterOfMass=Wheel_Loader.bodyGroups(27).subGroups(1).inertialProperties.centerOfMass+[0 0.831121913187700 -0.115829926648601]'*1e-5  CenterOfMassUnits=m  MomentsOfInertia=Wheel_Loader.bodyGroups(27).subGroups(1).inertialProperties.momentsOfInertia  MomentsOfInertiaUnits=kg*m^2  ProductsOfInertia=Wheel_Loader.bodyGroups(27).subGroups(1).inertialProperties.productsOfInertia  ProductsOfInertiaUnits=kg*m^2  GraphicType=FromGeometry  MarkerShape=Sphere  MarkerSize=10  GraphicVisPropType=SimpleVisualProperties  GraphicDiffuseColor=Wheel_Loader.bodyGroups(27).subGroups(1).visualProperties.rgb  GraphicOpacity=Wheel_Loader.bodyGroups(27).subGroups(1).visualProperties.opacity  GraphicSpecularColor=[0.5 0.5 0.5 1.0]  GraphicAmbientColor=[0.15 0.15 0.15 1.0]  GraphicEmissiveColor=[0.0 0.0 0.0 1.0]  GraphicShininess=75  DoExposeReferenceFrame=on  SerializedFrames=<Frames/>
  B1 : PMIOPort  Side=Left
  B2 : PMIOPort  Port=2  Side=Right
  connections:
  RT_Gnd_LRTire/RConn1 -- B2/RConn1
  RT_LR_WheelHub_Tire_Weld/RConn1 -- B1/RConn1
  Tire/RConn1 -- RT_LR_WheelHub_Tire_Weld/LConn1 -- RT_Gnd_LRTire/LConn1

== system sm_wheel_loader_lib/Wheel Loader Vehicle/Driveline/Wheel RR/Hub ==
  Bolts : sm_lib/Body Elements/File Solid  ExtGeomFileName=WheelRR_Hub_Bolts.STEP  UnitType=FromFile  ExtGeomFileUnits=m  StepReaderType=HEX  ExportConvexHullGeometry=off  InertiaType=Custom  BasedOnType=DensityFromFile  Density=1000  DensityUnits=kg/m^3  Mass=Wheel_Loader.bodyGroups(34).subGroups(2).inertialProperties.mass  MassUnits=kg  CenterOfMass=Wheel_Loader.bodyGroups(34).subGroups(2).inertialProperties.centerOfMass  CenterOfMassUnits=m  MomentsOfInertia=Wheel_Loader.bodyGroups(34).subGroups(2).inertialProperties.momentsOfInertia  MomentsOfInertiaUnits=kg*m^2  ProductsOfInertia=Wheel_Loader.bodyGroups(34).subGroups(2).inertialProperties.productsOfInertia  ProductsOfInertiaUnits=kg*m^2  GraphicType=FromGeometry  MarkerShape=Sphere  MarkerSize=10  GraphicVisPropType=SimpleVisualProperties  GraphicDiffuseColor=Wheel_Loader.bodyGroups(34).subGroups(2).visualProperties.rgb  GraphicOpacity=Wheel_Loader.bodyGroups(34).subGroups(2).visualProperties.opacity  GraphicSpecularColor=[0.5 0.5 0.5 1.0]  GraphicAmbientColor=[0.15 0.15 0.15 1.0]  GraphicEmissiveColor=[0.0 0.0 0.0 1.0]  GraphicShininess=75  DoExposeReferenceFrame=on  SerializedFrames=<Frames/>
  Hub : sm_lib/Body Elements/File Solid  ExtGeomFileName=WheelRR_Hub.STEP  UnitType=FromFile  ExtGeomFileUnits=m  StepReaderType=HEX  ExportConvexHullGeometry=off  InertiaType=Custom  BasedOnType=DensityFromFile  Density=1000  DensityUnits=kg/m^3  Mass=Wheel_Loader.bodyGroups(34).subGroups(1).inertialProperties.mass  MassUnits=kg  CenterOfMass=Wheel_Loader.bodyGroups(34).subGroups(1).inertialProperties.centerOfMass  CenterOfMassUnits=m  MomentsOfInertia=Wheel_Loader.bodyGroups(34).subGroups(1).inertialProperties.momentsOfInertia  MomentsOfInertiaUnits=kg*m^2  ProductsOfInertia=Wheel_Loader.bodyGroups(34).subGroups(1).inertialProperties.productsOfInertia  ProductsOfInertiaUnits=kg*m^2  GraphicType=FromGeometry  MarkerShape=Sphere  MarkerSize=10  GraphicVisPropType=SimpleVisualProperties  GraphicDiffuseColor=Wheel_Loader.bodyGroups(34).subGroups(1).visualProperties.rgb  GraphicOpacity=Wheel_Loader.bodyGroups(34).subGroups(1).visualProperties.opacity  GraphicSpecularColor=[0.5 0.5 0.5 1.0]  GraphicAmbientColor=[0.15 0.15 0.15 1.0]  GraphicEmissiveColor=[0.0 0.0 0.0 1.0]  GraphicShininess=75  DoExposeReferenceFrame=on  SerializedFrames=<Frames/>
  RT_RRFDCarrier_RRWheelHub_Weld : sm_lib/Frames and Transforms/Rigid Transform  RotationMethod=RotationMatrix  FollAlignAxisA=+X  BaseAlignAxisA=+Y  FollAlignAxisB=+Y  BaseAlignAxisB=+Z  RotationStandardAxis=+Z  RotationAngle=0.0  RotationAngleUnits=deg  RotationArbitraryAxis=[0 0 1]  RotationSequenceAxes=FollowerAxes  RotationSequence=XYX  RotationSequenceAngles=[0 0 0]  RotationSequenceAnglesUnits=deg  RotationMatrix=Wheel_Loader.coordSys(58).transform.rotation  Quaternion=[1 0 0 0]  TranslationMethod=Cartesian  TranslationCartesianOffset=Wheel_Loader.coordSys(58).transform.translation  TranslationCartesianOffsetUnits=m  TranslationStandardAxis=+Z  TranslationStandardOffset=0  TranslationStandardOffsetUnits=m  TranslationROffset=0  TranslationROffsetUnits=m  TranslationThetaOffset=0  TranslationThetaOffsetUnits=deg  TranslationZOffset=0  TranslationZOffsetUnits=m
  RT_RR_WheelHub_Tire_Weld : sm_lib/Frames and Transforms/Rigid Transform  RotationMethod=RotationMatrix  FollAlignAxisA=+X  BaseAlignAxisA=+Y  FollAlignAxisB=+Y  BaseAlignAxisB=+Z  RotationStandardAxis=+Z  RotationAngle=0.0  RotationAngleUnits=deg  RotationArbitraryAxis=[0 0 1]  RotationSequenceAxes=FollowerAxes  RotationSequence=XYX  RotationSequenceAngles=[0 0 0]  RotationSequenceAnglesUnits=deg  RotationMatrix=Wheel_Loader.coordSys(42).transform.rotation  Quaternion=[1 0 0 0]  TranslationMethod=Cartesian  TranslationCartesianOffset=Wheel_Loader.coordSys(42).transform.translation  TranslationCartesianOffsetUnits=m  TranslationStandardAxis=+Z  TranslationStandardOffset=0  TranslationStandardOffsetUnits=m  TranslationROffset=0  TranslationROffsetUnits=m  TranslationThetaOffset=0  TranslationThetaOffsetUnits=deg  TranslationZOffset=0  TranslationZOffsetUnits=m
  Rigid Transform : sm_lib/Frames and Transforms/Rigid Transform  RotationMethod=None  FollAlignAxisA=+X  BaseAlignAxisA=+Y  FollAlignAxisB=+Y  BaseAlignAxisB=+Z  RotationStandardAxis=+Z  RotationAngle=0.0  RotationAngleUnits=deg  RotationArbitraryAxis=[0 0 1]  RotationSequenceAxes=FollowerAxes  RotationSequence=XYX  RotationSequenceAngles=[0 0 0]  RotationSequenceAnglesUnits=deg  RotationMatrix=[1 0 0; 0 1 0; 0 0 1]  Quaternion=[1 0 0 0]  TranslationMethod=Cartesian  TranslationCartesianOffset="-[-0.000001665572481  -0.000009804046632 0]"  TranslationCartesianOffsetUnits=m  TranslationStandardAxis=+Z  TranslationStandardOffset=0  TranslationStandardOffsetUnits=m  TranslationROffset=0  TranslationROffsetUnits=m  TranslationThetaOffset=0  TranslationThetaOffsetUnits=deg  TranslationZOffset=0  TranslationZOffsetUnits=m
  B1 : PMIOPort  Side=Left
  F1 : PMIOPort  Port=2  Side=Right
  connections:
  Rigid Transform/RConn1 -- F1/RConn1
  RT_RRFDCarrier_RRWheelHub_Weld/RConn1 -- B1/RConn1
  RT_RR_WheelHub_Tire_Weld/LConn1 -- RT_RRFDCarrier_RRWheelHub_Weld/LConn1 -- Hub/RConn1 -- Bolts/RConn1
  RT_RR_WheelHub_Tire_Weld/RConn1 -- Rigid Transform/LConn1

== system sm_wheel_loader_lib/Wheel Loader Vehicle/Driveline/Wheel RR/Tire ==
  RT_Gnd_RRTire : sm_lib/Frames and Transforms/Rigid Transform  RotationMethod=RotationMatrix  FollAlignAxisA=+X  BaseAlignAxisA=+Y  FollAlignAxisB=+Y  BaseAlignAxisB=+Z  RotationStandardAxis=+Z  RotationAngle=0.0  RotationAngleUnits=deg  RotationArbitraryAxis=[0 0 1]  RotationSequenceAxes=FollowerAxes  RotationSequence=XYX  RotationSequenceAngles=[0 0 0]  RotationSequenceAnglesUnits=deg  RotationMatrix=Wheel_Loader.coordSys(42).transform.rotation  Quaternion=[1 0 0 0]  TranslationMethod=Cartesian  TranslationCartesianOffset=Wheel_Loader.coordSys(42).transform.translation  TranslationCartesianOffsetUnits=m  TranslationStandardAxis=+Z  TranslationStandardOffset=0  TranslationStandardOffsetUnits=m  TranslationROffset=0  TranslationROffsetUnits=m  TranslationThetaOffset=0  TranslationThetaOffsetUnits=deg  TranslationZOffset=0  TranslationZOffsetUnits=m
  RT_RR_WheelHub_Tire_Weld : sm_lib/Frames and Transforms/Rigid Transform  RotationMethod=RotationMatrix  FollAlignAxisA=+X  BaseAlignAxisA=+Y  FollAlignAxisB=+Y  BaseAlignAxisB=+Z  RotationStandardAxis=+Z  RotationAngle=0.0  RotationAngleUnits=deg  RotationArbitraryAxis=[0 0 1]  RotationSequenceAxes=FollowerAxes  RotationSequence=XYX  RotationSequenceAngles=[0 0 0]  RotationSequenceAnglesUnits=deg  RotationMatrix=Wheel_Loader.coordSys(42).transform.rotation  Quaternion=[1 0 0 0]  TranslationMethod=Cartesian  TranslationCartesianOffset=Wheel_Loader.coordSys(42).transform.translation  TranslationCartesianOffsetUnits=m  TranslationStandardAxis=+Z  TranslationStandardOffset=0  TranslationStandardOffsetUnits=m  TranslationROffset=0  TranslationROffsetUnits=m  TranslationThetaOffset=0  TranslationThetaOffsetUnits=deg  TranslationZOffset=0  TranslationZOffsetUnits=m
  Tire : sm_lib/Body Elements/File Solid  ExtGeomFileName=WheelRR_Tire.STEP  UnitType=FromFile  ExtGeomFileUnits=m  StepReaderType=HEX  ExportConvexHullGeometry=off  InertiaType=Custom  BasedOnType=DensityFromFile  Density=1000  DensityUnits=kg/m^3  Mass=Wheel_Loader.bodyGroups(26).subGroups(1).inertialProperties.mass  MassUnits=kg  CenterOfMass=Wheel_Loader.bodyGroups(26).subGroups(1).inertialProperties.centerOfMass+[0 0.826059194754229 -0.192329590465679]'*1.0e-05  CenterOfMassUnits=m  MomentsOfInertia=Wheel_Loader.bodyGroups(26).subGroups(1).inertialProperties.momentsOfInertia  MomentsOfInertiaUnits=kg*m^2  ProductsOfInertia=Wheel_Loader.bodyGroups(26).subGroups(1).inertialProperties.productsOfInertia  ProductsOfInertiaUnits=kg*m^2  GraphicType=FromGeometry  MarkerShape=Sphere  MarkerSize=10  GraphicVisPropType=SimpleVisualProperties  GraphicDiffuseColor=Wheel_Loader.bodyGroups(26).subGroups(1).visualProperties.rgb  GraphicOpacity=Wheel_Loader.bodyGroups(26).subGroups(1).visualProperties.opacity  GraphicSpecularColor=[0.5 0.5 0.5 1.0]  GraphicAmbientColor=[0.15 0.15 0.15 1.0]  GraphicEmissiveColor=[0.0 0.0 0.0 1.0]  GraphicShininess=75  DoExposeReferenceFrame=on  SerializedFrames=<Frames/>
  B1 : PMIOPort  Side=Left
  B2 : PMIOPort  Port=2  Side=Right
  connections:
  RT_Gnd_RRTire/LConn1 -- RT_RR_WheelHub_Tire_Weld/LConn1 -- Tire/RConn1
  RT_RR_WheelHub_Tire_Weld/RConn1 -- B1/RConn1
  RT_Gnd_RRTire/RConn1 -- B2/RConn1
